simulink model "lab1_smirnov_simulink"  (R2023a)
settings: Solver=FixedStepDiscrete  StartTime=0.0  StopTime=10.0  FixedStep=0.001  RelTol=1e-3
libraries: simulink x1
settings Model: Creator=maybn  LastModifiedBy=maybn

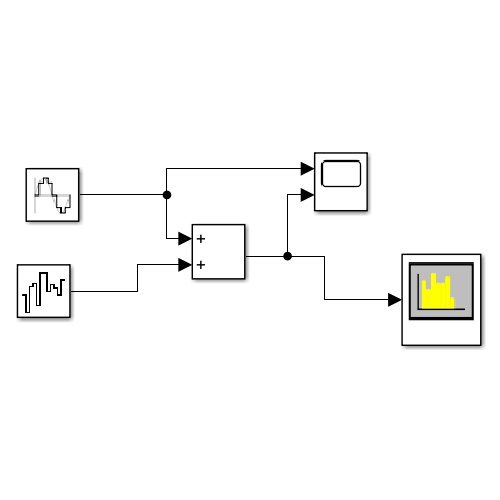
[thumbnail: Simulink's stored preview of the top-level diagram]
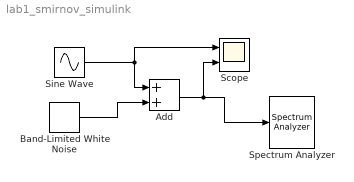
== system lab1_smirnov_simulink ==
  Add : Sum
  Band-Limited White Noise : simulink/Sources/Band-Limited White Noise  Cov=[0.1]  Ts=0.1  seed=[23341]
  Scope : Scope  NumInputPorts=2
  Sine Wave : Sin  SampleTime=0.001
  Spectrum Analyzer : SpectrumAnalyzer  WindowPosition=[265.000000,144.000000,800.000000,526.000000,]  ScopeFrameLocation=window  Span=1000  StartFrequency=-500  StopFrequency=500  YLimits=[-53.04249587,31.26153144]  ColorLimits=[-80 20]  SelectedToolstripTab=spectrumAnalyzerToolstrip.estimationTab
  wires:
  Sine Wave/1 -> Add/1, Scope/1
  Band-Limited White Noise/1 -> Add/2
  Add/1 -> Scope/2, Spectrum Analyzer/1
